simulink model "robotics_coursework_simulation"  (R2025b)
settings: Solver=VariableStepAuto  StartTime=0.0  StopTime=10.0  RelTol=1e-3
undefined symbols (not defined in the file): K, mu, mu1, tou
settings Model: Creator=javve  LastModifiedBy=javve

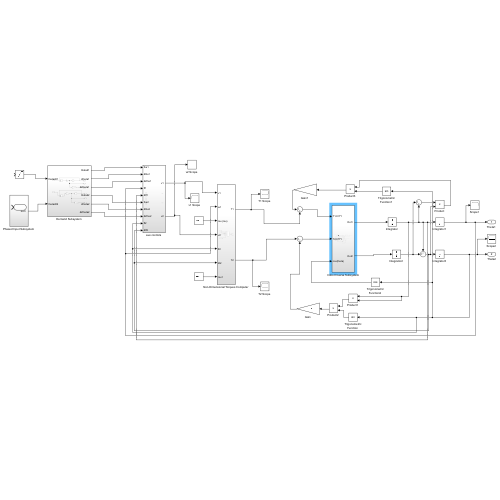
[thumbnail: Simulink's stored preview of the top-level diagram]
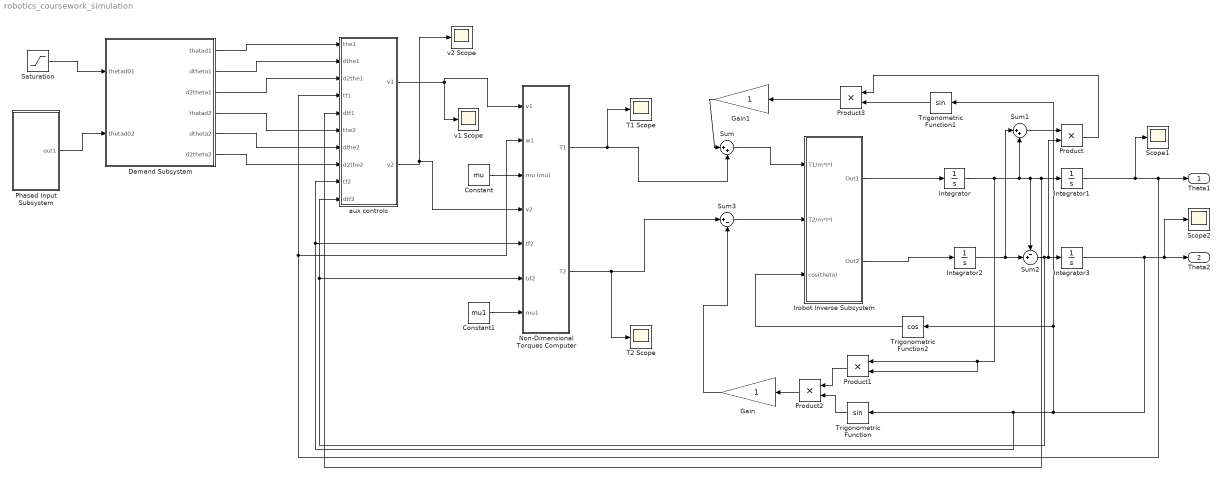
== system robotics_coursework_simulation ==
  Constant : Constant  Value=mu
  Constant1 : Constant  Value=mu1
  "Demand Subsystem " : Subsystem
  "Gain " : Gain
  "Gain1  " : Gain
  "Integrator " : Integrator
  "Integrator1 " : Integrator
  "Integrator2 " : Integrator
  "Integrator3 " : Integrator
  Irobot Inverse Subsystem : Subsystem
  "Non-Dimensional Torques Computer " : Subsystem
  "Phased Input Subsystem " : Subsystem
  "Product " : Product
  "Product1 " : Product
  "Product2 " : Product
  "Product3 " : Product
  Saturation : Saturate
  "Scope1 " : Scope
  "Scope2 " : Scope
  Sum : Sum  Inputs=|++
  Sum1 : Sum  Inputs=|++
  Sum2 : Sum  Inputs=-+|
  Sum3 : Sum  Inputs=|+-
  "T1 Scope " : Scope
      settings: DataLoggingVariableName=ScopeData2
  "T2 Scope " : Scope
      settings: DataLoggingVariableName=ScopeData3
  "Trigonometric Function " : Trigonometry
  "Trigonometric Function1 " : Trigonometry
  "Trigonometric Function2 " : Trigonometry  Operator=cos
  "aux controls " : Subsystem
  "v1 Scope " : Scope
      settings: DataLoggingVariableName=ScopeData4
  "v2 Scope " : Scope
      settings: DataLoggingVariableName=ScopeData5
  "Theta1 " : Outport
  Theta2 : Outport  Port=2
  wires:
  "Gain1  "/1 -> Sum/1
  "Product3 "/1 -> "Gain1  "/1
  "Trigonometric Function1 "/1 -> "Product3 "/2
  "Product "/1 -> "Product3 "/1
  "Non-Dimensional Torques Computer "/1("T1 ") -> "T1 Scope "/1, Sum/2
  Sum1/1 -> "Product "/1
  "Product1 "/1 -> "Product2 "/1
  "Trigonometric Function "/1 -> "Product2 "/2
  Irobot Inverse Subsystem/2("Out2 ") -> "Integrator2 "/1
  Irobot Inverse Subsystem/1("Out1 ") -> "Integrator "/1
  "Trigonometric Function2 "/1 -> Irobot Inverse Subsystem/3(cos(theta))
  Sum/1 -> Irobot Inverse Subsystem/1(T1/m*I*I)
  "Integrator2 "/1 -> Sum1/1, Sum2/2
  "Non-Dimensional Torques Computer "/2("T2 ") -> "T2 Scope "/1, Sum3/1
  Sum3/1 -> Irobot Inverse Subsystem/2(T2/m*I*I)
  "Gain "/1 -> Sum3/2
  "Product2 "/1 -> "Gain "/1
  Constant/1 -> "Non-Dimensional Torques Computer "/3(mu (mu))
  "aux controls "/1("v1 ") -> "Non-Dimensional Torques Computer "/1("v1 "), "v1 Scope "/1
  "aux controls "/2("v2 ") -> "v2 Scope "/1, "Non-Dimensional Torques Computer "/4("v2 ")
  Constant1/1 -> "Non-Dimensional Torques Computer "/7("mu1 ")
  "Demand Subsystem "/6("d2theta2 ") -> "aux controls "/8("d2the2 ")
  "Demand Subsystem "/5("dtheta2 ") -> "aux controls "/7("dthe2 ")
  "Demand Subsystem "/4("thatad2 ") -> "aux controls "/6("the2 ")
  "Demand Subsystem "/3("d2theta1 ") -> "aux controls "/3("d2the1 ")
  "Demand Subsystem "/2("dtheta1 ") -> "aux controls "/2("dthe1 ")
  "Demand Subsystem "/1("thatad1 ") -> "aux controls "/1("the1 ")
  Saturation/1 -> "Demand Subsystem "/1("thetad01 ")
  "Integrator1 "/1 -> "Scope1 "/1, "Non-Dimensional Torques Computer "/2("w1 "), "aux controls "/4("tf1 "), "Theta1 "/1
  "Integrator "/1 -> "Product1 "/1, "Product1 "/2, Sum1/2, Sum2/1, "aux controls "/5("dtf1 "), "Integrator1 "/1
  "Integrator3 "/1 -> "Trigonometric Function1 "/1, "Trigonometric Function2 "/1, "Non-Dimensional Torques Computer "/5("tf2 "), "aux controls "/9("tf2 "), "Trigonometric Function "/1, "Scope2 "/1, Theta2/1
  Sum2/1 -> "Non-Dimensional Torques Computer "/6("td2 "), "aux controls "/10("dtf2 "), "Product "/2, "Integrator3 "/1
  "Phased Input Subsystem "/1("out1  ") -> "Demand Subsystem "/2("thetad02 ")

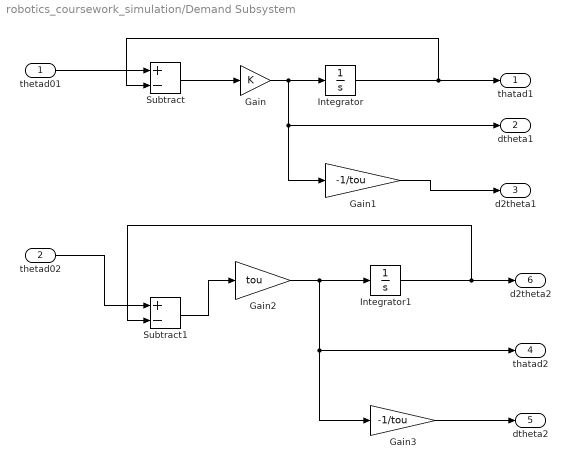
== system robotics_coursework_simulation/Demand Subsystem  ==
  "thetad01 " : Inport
  "thetad02 " : Inport  Port=2
  Gain : Gain  Gain=K
  Gain1 : Gain  Gain=-1/tou
  Gain2 : Gain  Gain=tou
  Gain3 : Gain  Gain=-1/tou
  Integrator : Integrator
  Integrator1 : Integrator
  Subtract : Sum  Inputs=+-
  Subtract1 : Sum  Inputs=+-
  "thatad1 " : Outport
  "dtheta1 " : Outport  Port=2
  "d2theta1 " : Outport  Port=3
  "thatad2 " : Outport  Port=4
  "dtheta2 " : Outport  Port=5
  "d2theta2 " : Outport  Port=6
  wires:
  "thetad01 "/1 -> Subtract/1
  Subtract/1 -> Gain/1
  Gain/1 -> "dtheta1 "/1, Gain1/1, Integrator/1
  Integrator/1 -> Subtract/2, "thatad1 "/1
  Gain1/1 -> "d2theta1 "/1
  "thetad02 "/1 -> Subtract1/1
  Subtract1/1 -> Gain2/1
  Gain2/1 -> "thatad2 "/1, Gain3/1, Integrator1/1
  Integrator1/1 -> Subtract1/2, "d2theta2 "/1
  Gain3/1 -> "dtheta2 "/1

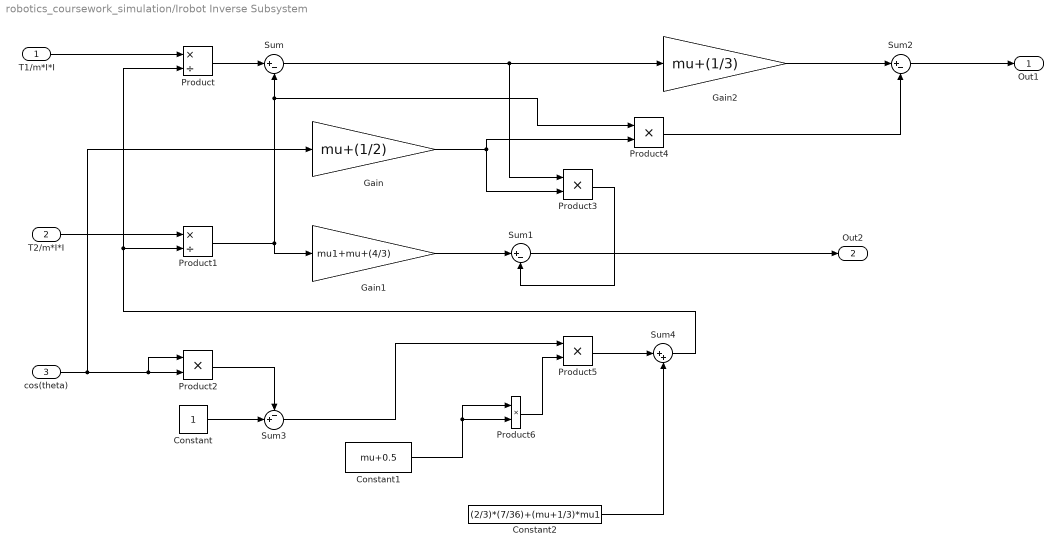
== system robotics_coursework_simulation/Irobot Inverse Subsystem ==
  T1/m*I*I : Inport
  T2/m*I*I : Inport  Port=2
  cos(theta) : Inport  Port=3
  Constant : Constant
  Constant1 : Constant  Value=mu+0.5
  Constant2 : Constant  Value=(2/3)*(7/36)+(mu+1/3)*mu1
  Gain : Gain  Gain=mu+(1/2)
  Gain1 : Gain  Gain=mu1+mu+(4/3)
  Gain2 : Gain  Gain=mu+(1/3)
  Product : Product  Inputs=*/
  Product1 : Product  Inputs=*/
  Product{2..6} (5 alike) : Product
  Sum : Sum  Inputs=|+-
  Sum1 : Sum  Inputs=|+-
  Sum2 : Sum  Inputs=|+-
  Sum3 : Sum  Inputs=-+|
  Sum4 : Sum  Inputs=|++
  "Out1 " : Outport
  "Out2 " : Outport  Port=2
  wires:
  T1/m*I*I/1 -> Product/1
  T2/m*I*I/1 -> Product1/1
  cos(theta)/1 -> Product2/1, Product2/2, Gain/1
  Gain/1 -> Product4/2, Product3/2
  Product/1 -> Sum/1
  Product1/1 -> Product4/1, Sum/2, Gain1/1
  Sum/1 -> Gain2/1, Product3/1
  Gain1/1 -> Sum1/1
  Sum1/1 -> "Out2 "/1
  Product3/1 -> Sum1/2
  Gain2/1 -> Sum2/1
  Product4/1 -> Sum2/2
  Sum2/1 -> "Out1 "/1
  Product2/1 -> Sum3/1
  Constant/1 -> Sum3/2
  Sum3/1 -> Product5/1
  Constant1/1 -> Product6/1, Product6/2
  Product6/1 -> Product5/2
  Product5/1 -> Sum4/1
  Constant2/1 -> Sum4/2
  Sum4/1 -> Product1/2, Product/2

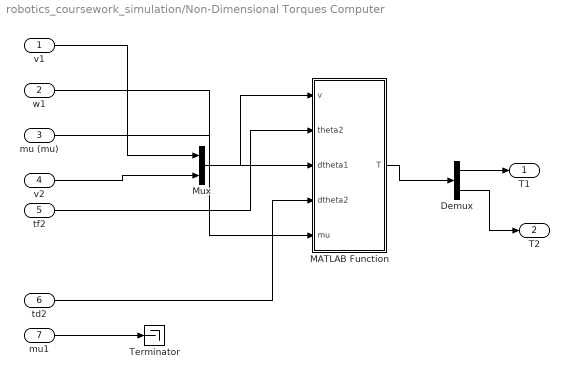
== system robotics_coursework_simulation/Non-Dimensional Torques Computer  ==
  "v1 " : Inport
  "w1 " : Inport  Port=2
  mu (mu) : Inport  Port=3
  "v2 " : Inport  Port=4
  "tf2 " : Inport  Port=5
  "td2 " : Inport  Port=6
  "mu1 " : Inport  Port=7
  Demux : Demux  Outputs=2
  MATLAB Function : MATLAB Function  TreatAsAtomicUnit=on
  Mux : Mux  Inputs=2
  Terminator : Terminator
  "T1 " : Outport
  "T2 " : Outport  Port=2
  wires:
  "v1 "/1 -> Mux/1
  "w1 "/1 -> MATLAB Function/3(dtheta1)
  "v2 "/1 -> Mux/2
  Mux/1 -> MATLAB Function/1(v)
  "tf2 "/1 -> MATLAB Function/2(theta2)
  "td2 "/1 -> MATLAB Function/4(dtheta2)
  mu (mu)/1 -> MATLAB Function/5(mu)
  MATLAB Function/1(T) -> Demux/1
  Demux/1 -> "T1 "/1
  Demux/2 -> "T2 "/1
  "mu1 "/1 -> Terminator/1

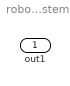
== system robotics_coursework_simulation/Phased Input Subsystem  ==
  "out1  " : Outport

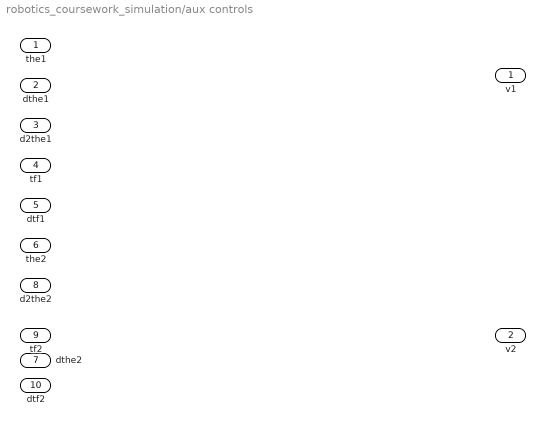
== system robotics_coursework_simulation/aux controls  ==
  "the1 " : Inport
  "dthe1 " : Inport  Port=2
  "d2the1 " : Inport  Port=3
  "tf1 " : Inport  Port=4
  "dtf1 " : Inport  Port=5
  "the2 " : Inport  Port=6
  "dthe2 " : Inport  Port=7
  "d2the2 " : Inport  Port=8
  "tf2 " : Inport  Port=9
  "dtf2 " : Inport  Port=10
  "v1 " : Outport
  "v2 " : Outport  Port=2

== matlab function robotics_coursework_simulation/Non-Dimensional Torques Computer /MATLAB Function ==
  data: v input; T output; theta2 input; dtheta1 input; dtheta2 input; mu input
function T = nondim_torque(v, theta2, dtheta1, dtheta2, mu)
% Non-dimensional torque computation for 2-link arm

v1 = v(1);
v2 = v(2);

% ----- Inertia matrix M* -----
I11 = 1 + mu + 2*mu*cos(theta2);
I12 = mu*cos(theta2) + mu/2;
I21 = I12;
I22 = mu/2;

% ----- Coriolis / centrifugal -----
C1 = -mu*(2*dtheta1*dtheta2 + dtheta2^2)*sin(theta2);
C2 =  mu*(dtheta1^2)*sin(theta2);

% ----- Torques -----
T1 = I11*v1 + I12*v2 + C1;
T2 = I21*v1 + I22*v2 + C2;

T = [T1; T2];
end
